simulink model "simscape1j"  (R2025b)
settings: Solver=ode15s  StartTime=0.0  StopTime=100  RelTol=1e-3  AbsTol=1e-3
values from neighbouring files (symbols this model uses):
  g = 32.174    [RCSMasterCalcs.m]    (also in RCS_180_sweep.m)
  Ixxp = 252099.557 * 0.00029263965    (= 73.7743261256)    [ParabolicNozzle.m]    (also in RCSMasterCalcs.m = 54.4132332957; RCS_180_sweep.m = 12.6144279283)
  mdot_slugs = (Cd * A_actual_m2 * P0_Pa * choke / 0.4536) / g    [RCS_180_sweep.m]
  r_nozzle = 5.0 / 12.0    (= 0.416666666667)    [RCS_180_sweep.m]
libraries: fl_lib x18, nesl_utility x8, ee_lib x2
settings Model: Creator=Lana  LastModifiedBy=Lana
settings SolverCC: AutoScaleAbsTol=off  AlgebraicLoopSolver=TrustRegion  MaxZcPerStep=1.0
settings DebuggingCC: UnconnectedInputMsg=warning  UnconnectedOutputMsg=warning  UnconnectedLineMsg=warning  SymbolicDimsDataTypeCodeGenerationDiagnostic=none
settings ModelReferenceCC: EnableRefExpFcnMdlSchedulingChecks=on
settings SFSimCC: CustomCodeUndefinedFunction=UseInterfaceOnly
settings RTWCC: GPUComputeCapability=3.5  DLArmComputeVersion=19.05
settings SimscapeCC: SimscapeLogType=all  SimscapeLogSimulationStatistics=on  SimscapeLogDataHistory=10000.0

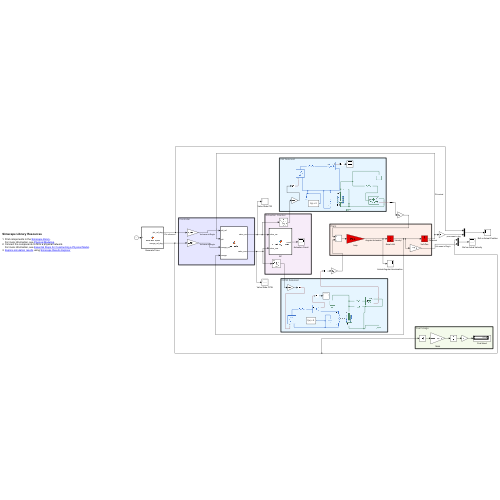
[thumbnail: Simulink's stored preview of the top-level diagram]
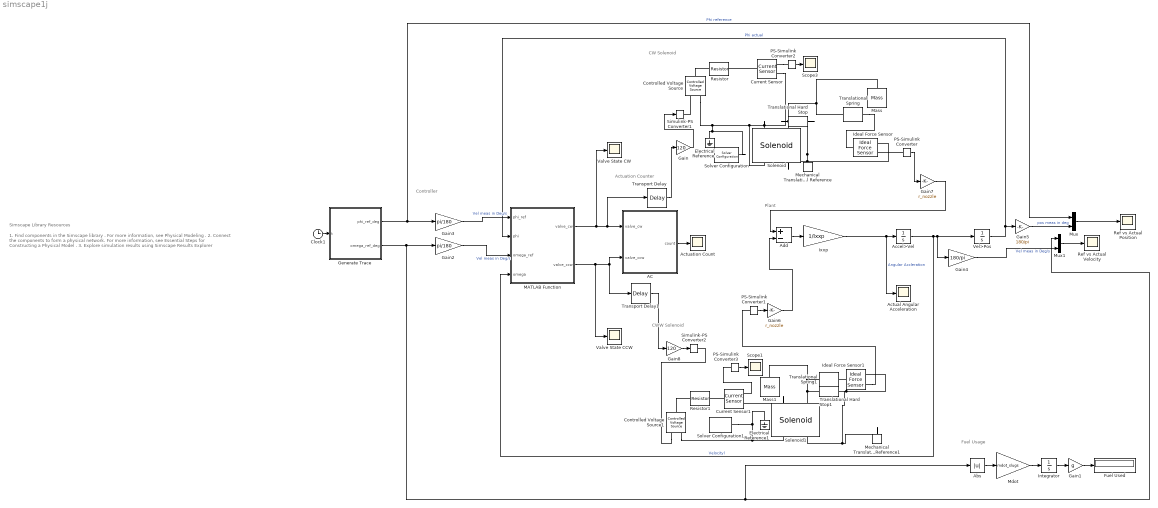
== system simscape1j ==
  note: 1. Find components in the Simscape library .
      | For more information, see Physical Modeling .
      | 2. Connect the components to form a physical network.
      | For more information, see Essential Steps for Constructing a Physical Model .
      | 3. Explore simulation results using Simscape Results Explorer
  note: Simscape Library Resources
  note: Controller
  note: CW Solenoid
  note: Plant
  note: Fuel Usage
  note: Actuation Counter
  note: CWW Solenoid
  AC : MATLAB Function  TreatAsAtomicUnit=on
  Abs : Abs  SaturateOnIntegerOverflow=off
  Accel>Vel : Integrator
  "Actual Angular Acceleration " : Scope
      settings: ActiveDisplayYMinimum=-10.034483776335616  ActiveDisplayYMaximum=37.904655593220141  DataLoggingVariableName=ScopeData4
  Actuation Count : Scope
      settings: ActiveDisplayYMinimum=-1.4453272832049562  ActiveDisplayYMaximum=5.9313739118884694  DataLoggingVariableName=ScopeData3
  Add : Sum  Inputs=+-
  Clock1 : Clock
  Controlled Voltage Source : fl_lib/Electrical/Electrical Sources/Controlled Voltage Source
  Controlled Voltage Source1 : fl_lib/Electrical/Electrical Sources/Controlled Voltage Source
  Current Sensor : fl_lib/Electrical/Electrical Sensors/Current Sensor
  Current Sensor1 : fl_lib/Electrical/Electrical Sensors/Current Sensor
  Electrical Reference : fl_lib/Electrical/Electrical Elements/Electrical Reference
  Electrical Reference1 : fl_lib/Electrical/Electrical Elements/Electrical Reference
  Fuel Used : Display
  Gain : Gain  Gain=120
  Gain1 : Gain  Gain=g
  Gain2 : Gain  Gain=pi/180
  Gain3 : Gain  Gain=pi/180
  Gain4 : Gain  Gain=180/pi
  Gain5 : Gain  Gain=180/pi
  Gain6 : Gain  Gain=r_nozzle
  Gain7 : Gain  Gain=r_nozzle
  Gain8 : Gain  Gain=120
  Generate Trace : MATLAB Function  TreatAsAtomicUnit=on
  Ideal Force Sensor : fl_lib/Mechanical/Mechanical Sensors/Ideal Force Sensor
  Ideal Force Sensor1 : fl_lib/Mechanical/Mechanical Sensors/Ideal Force Sensor
  Integrator : Integrator
  Ixxp : Gain  Gain=1/Ixxp
  MATLAB Function : MATLAB Function  TreatAsAtomicUnit=on  SystemSampleTime=0.005
  Mass : fl_lib/Mechanical/Translational Elements/Mass  mass=0.05 kg  num_ports=foundation.enum.numPorts2.one  v_specify=off  v_priority=High  v=0 m/s  v_nominal_specify=off  v_nominal_value=1  v_nominal_unit=m/s  f_specify=off  f_priority=None  f=0 N  f_nominal_specify=off  f_nominal_value=1  f_nominal_unit=N
  Mass1 : fl_lib/Mechanical/Translational Elements/Mass  mass=0.05 kg  num_ports=foundation.enum.numPorts2.one  v_specify=off  v_priority=High  v=0 m/s  v_nominal_specify=off  v_nominal_value=1  v_nominal_unit=m/s  f_specify=off  f_priority=None  f=0 N  f_nominal_specify=off  f_nominal_value=1  f_nominal_unit=N
  Mdot : Gain  Gain=mdot_slugs
  Mechanical Translational Reference : fl_lib/Mechanical/Translational Elements/Mechanical Translational Reference
  Mechanical Translational Reference1 : fl_lib/Mechanical/Translational Elements/Mechanical Translational Reference
  Mux : Mux  Inputs=2
  Mux1 : Mux  Inputs=2
  PS-Simulink Converter{,1..3} (4 alike) : nesl_utility/PS-Simulink Converter  PhysicalDomain=network_engine_domain  SubClassName=ps_output  LeftPortType=input  RightPortType=output  PseudoPeriodic=off  Frequencies=[]  VectorFormat=inherit  Unit=inherit  AffineConversion=off
  Ref vs Actual Position : Scope
      settings: ActiveDisplayYMinimum=-22.500002652240926  ActiveDisplayYMaximum=202.50000029469345  DataLoggingVariableName=ScopeData5
  Ref vs Actual Velocity : Scope
      settings: ActiveDisplayYMinimum=-4.4232598731139454  ActiveDisplayYMaximum=10.223921060317231
  Resistor : fl_lib/Electrical/Electrical Elements/Resistor  R=1200 Ohm  i_specify=off  i_priority=None  i=0 A  i_nominal_specify=off  i_nominal_value=1  i_nominal_unit=A  v_specify=off  v_priority=None  v=0 V  v_nominal_specify=off  v_nominal_value=1  v_nominal_unit=V
  Resistor1 : fl_lib/Electrical/Electrical Elements/Resistor  R=1200 Ohm  i_specify=off  i_priority=None  i=0 A  i_nominal_specify=off  i_nominal_value=1  i_nominal_unit=A  v_specify=off  v_priority=None  v=0 V  v_nominal_specify=off  v_nominal_value=1  v_nominal_unit=V
  Scope1 : Scope
      settings: ActiveDisplayYMinimum=-0.01250008529219436  ActiveDisplayYMaximum=0.11250076762974927  DataLoggingVariableName=ScopeData2
  Scope3 : Scope
      settings: ActiveDisplayYMinimum=-0.01250008529219436  ActiveDisplayYMaximum=0.11250076762974927  DataLoggingVariableName=ScopeData8
  Simulink-PS Converter1 : nesl_utility/Simulink-PS Converter  PhysicalDomain=network_engine_domain  SubClassName=ps_input  LeftPortType=input  RightPortType=output  PseudoPeriodic=off  Frequencies=[]  NoiseDistribution=none  NoiseParameters=[]  Unit=1  AffineConversion=off  FilteringAndDerivatives=filter  SimscapeFilterOrder=1  InputFilterTimeConstant=0.001  UdotUserProvided=0
  Simulink-PS Converter2 : nesl_utility/Simulink-PS Converter  PhysicalDomain=network_engine_domain  SubClassName=ps_input  LeftPortType=input  RightPortType=output  PseudoPeriodic=off  Frequencies=[]  NoiseDistribution=none  NoiseParameters=[]  Unit=1  AffineConversion=off  FilteringAndDerivatives=filter  SimscapeFilterOrder=1  InputFilterTimeConstant=0.001  UdotUserProvided=0
  Solenoid : ee_lib/Electromechanical/Mechatronic Actuators/Solenoid  motionDirection=ee.enum.actuators.solenoidDirection.towards  F12=[100, 45] N  X12=[0.1, 1.5] mm  Vdc=120 V  Imax=0.133 A  K=25000 N/m  Xzero=0 mm  lam=50 N*s/m  Mass=0.08 kg  Xmax=5 mm  K_endstop=1e8 N/m  D_endstop=500 N*s/m  i_specify=on  i_priority=Low  i=0 A  i_nominal_specify=off  i_nominal_value=0.1  i_nominal_unit=A  x_specify=on  x_priority=Low  x=0.1 mm  x_nominal_specify=off  x_nominal_value=1  x_nominal_unit=mm  vel_specify=on  vel_priority=High  vel=0 mm/s  vel_nominal_specify=off  vel_nominal_value=1  vel_nominal_unit=mm/s  F_specify=on  F_priority=High  F=0 N  F_nominal_specify=off  F_nominal_value=100  F_nominal_unit=N  v_L_specify=off  v_L_priority=None  v_L=0 V  v_L_nominal_specify=off  v_L_nominal_value=1  v_L_nominal_unit=V  magnetic_force_specify=off  magnetic_force_priority=None  magnetic_force=0 N  magnetic_force_nominal_specify=off  magnetic_force_nominal_value=1  magnetic_force_nominal_unit=N  alpha=3.93e-3 1/K  Tmeas=25 degC  thermal_mass=100 J/K  temperature_specify=off  temperature_priority=High  temperature=25 degC  temperature_nominal_specify=off  temperature_nominal_value=1  temperature_nominal_unit=degC  Q_specify=off  Q_priority=None  Q=0 W  Q_nominal_specify=off  Q_nominal_value=1  Q_nominal_unit=W
      settings: InternalSimscapePortConfiguration="{\"Bottom\":[],\"Left\":[{\"id\":\"p\",\"label\":\"+\",\"type\":\"foundation.electrical.electrical\"},{\"id\":\"R\",\"label\":\"R\",\"type\":\"foundation.mechanical.translational.translational\"}],\"Right\":[{\"id\":\"n\",\"label\":\"-\",\"type\":\"foundation.electrical.electrical\"},{\"id\":\"C\",\"label\":\"C\",\"type\":\"foundation.mechanical.translational.translational\"}],\"Top\":[]}"
  Solenoid1 : ee_lib/Electromechanical/Mechatronic Actuators/Solenoid  motionDirection=ee.enum.actuators.solenoidDirection.towards  F12=[100, 45] N  X12=[0.1, 1.5] mm  Vdc=120 V  Imax=0.133 A  K=25000 N/m  Xzero=0 mm  lam=50 N*s/m  Mass=0.08 kg  Xmax=5 mm  K_endstop=1e8 N/m  D_endstop=500 N*s/m  i_specify=on  i_priority=Low  i=0 A  i_nominal_specify=off  i_nominal_value=1  i_nominal_unit=A  x_specify=on  x_priority=Low  x=0.1 mm  x_nominal_specify=off  x_nominal_value=1  x_nominal_unit=mm  vel_specify=on  vel_priority=High  vel=0 mm/s  vel_nominal_specify=off  vel_nominal_value=1  vel_nominal_unit=mm/s  F_specify=on  F_priority=High  F=0 N  F_nominal_specify=off  F_nominal_value=1  F_nominal_unit=N  v_L_specify=off  v_L_priority=None  v_L=0 V  v_L_nominal_specify=off  v_L_nominal_value=1  v_L_nominal_unit=V  magnetic_force_specify=off  magnetic_force_priority=None  magnetic_force=0 N  magnetic_force_nominal_specify=off  magnetic_force_nominal_value=1  magnetic_force_nominal_unit=N  alpha=3.93e-3 1/K  Tmeas=25 degC  thermal_mass=100 J/K  temperature_specify=off  temperature_priority=High  temperature=25 degC  temperature_nominal_specify=off  temperature_nominal_value=1  temperature_nominal_unit=degC  Q_specify=off  Q_priority=None  Q=0 W  Q_nominal_specify=off  Q_nominal_value=1  Q_nominal_unit=W
      settings: InternalSimscapePortConfiguration="{\"Bottom\":[],\"Left\":[{\"id\":\"p\",\"label\":\"+\",\"type\":\"foundation.electrical.electrical\"},{\"id\":\"R\",\"label\":\"R\",\"type\":\"foundation.mechanical.translational.translational\"}],\"Right\":[{\"id\":\"n\",\"label\":\"-\",\"type\":\"foundation.electrical.electrical\"},{\"id\":\"C\",\"label\":\"C\",\"type\":\"foundation.mechanical.translational.translational\"}],\"Top\":[]}"
  Solver Configuration : nesl_utility/Solver Configuration  PhysicalDomain=network_engine_domain  SubClassName=solver  LeftPortType=input  RightPortType=generic  Tones=[]  Harmonics=[]  SimulateNoise=off  Profile=off  UseLocalSampling=off  EnableSwitchedLinearOptims=on  FrequencyDomain=off  UseCCode=off  RelTol=0.001  AbsTol=0.001  MinStep=1e-09  ToWorkspace=off  RevertToSquareIcSolve=off  NumHomotopyIterations=100  PhasorMode=off  PhasorModeNumHarmonics=1  ConsistencySolver=NEWTON_XTOL_AFTER_FTOL  IndexReductionMethod=DerivativeReplacement  DoDC=off  ResidualTolerance=1e-09  ConsistencyTolSource=GLOBAL  ConsistencyAbsTol=0.001  ConsistencyRelTol=0.001  ConsistencyTolFactor=0.001  UseLocalSolver=off  LocalSolverChoice=NE_BACKWARD_EULER_ADVANCER  ResolveIndetEquations=on  FunctionEvalNumThread=1  LocalSolverSampleTime=0.001  DoFixedCost=off  MaxNonlinIter=3  MaxModeIter=2  ComputeImpulses=off  ImpulseIterations=2  LinearAlgebra=auto  LinearAlgebraNumThread=0  EquationFormulation=NE_TIME_EF  DelaysMemoryBudget=1024  AutomaticFiltering=on  FilteringTimeConstant=0.001  PartitionStorageMethod=AS_NEEDED  PartitionMemoryBudget=1024  PartitionMethod=ROBUST  MultibodyUseLocalSolver=off  MultibodyLocalSolverChoice=ODE1  MultibodyLocalSolverSampleTime=0.001
  Solver Configuration1 : nesl_utility/Solver Configuration  PhysicalDomain=network_engine_domain  SubClassName=solver  LeftPortType=input  RightPortType=generic  Tones=[]  Harmonics=[]  SimulateNoise=off  Profile=off  UseLocalSampling=off  EnableSwitchedLinearOptims=on  FrequencyDomain=off  UseCCode=off  RelTol=0.001  AbsTol=0.001  MinStep=1e-09  ToWorkspace=off  RevertToSquareIcSolve=off  NumHomotopyIterations=100  PhasorMode=off  PhasorModeNumHarmonics=1  ConsistencySolver=NEWTON_XTOL_AFTER_FTOL  IndexReductionMethod=DerivativeReplacement  DoDC=off  ResidualTolerance=1e-09  ConsistencyTolSource=GLOBAL  ConsistencyAbsTol=0.001  ConsistencyRelTol=0.001  ConsistencyTolFactor=0.001  UseLocalSolver=off  LocalSolverChoice=NE_BACKWARD_EULER_ADVANCER  ResolveIndetEquations=on  FunctionEvalNumThread=1  LocalSolverSampleTime=0.001  DoFixedCost=off  MaxNonlinIter=3  MaxModeIter=2  ComputeImpulses=off  ImpulseIterations=2  LinearAlgebra=auto  LinearAlgebraNumThread=0  EquationFormulation=NE_TIME_EF  DelaysMemoryBudget=1024  AutomaticFiltering=on  FilteringTimeConstant=0.001  PartitionStorageMethod=AS_NEEDED  PartitionMemoryBudget=1024  PartitionMethod=ROBUST  MultibodyUseLocalSolver=off  MultibodyLocalSolverChoice=ODE1  MultibodyLocalSolverSampleTime=0.001
  Translational Hard Stop : fl_lib/Mechanical/Translational Elements/Translational Hard Stop  upper_bnd=0.005 m  lower_bnd=-.0001 m  model=simscape.enum.hardstop.smooth  stiff_up=1e6 N/m  stiff_low=1e6 N/m  D_up=150 N*s/m  D_low=150 N*s/m  transition=0.1 mm  coeff_rest=0.7  v_tol=0.001 m/s  f_tol=0.001 N  v_specify=off  v_priority=None  v=0 m/s  v_nominal_specify=off  v_nominal_value=1  v_nominal_unit=m/s  f_specify=off  f_priority=None  f=0 N  f_nominal_specify=off  f_nominal_value=1  f_nominal_unit=N  x_specify=off  x_priority=High  x=0 m  x_nominal_specify=off  x_nominal_value=1  x_nominal_unit=m  M_specify=off  M_priority=None  M=0
  Translational Hard Stop1 : fl_lib/Mechanical/Translational Elements/Translational Hard Stop  upper_bnd=0.005 m  lower_bnd=-.0001 m  model=simscape.enum.hardstop.smooth  stiff_up=1e6 N/m  stiff_low=1e6 N/m  D_up=150 N*s/m  D_low=150 N*s/m  transition=0.1 mm  coeff_rest=0.7  v_tol=0.001 m/s  f_tol=0.001 N  v_specify=off  v_priority=None  v=0 m/s  v_nominal_specify=off  v_nominal_value=1  v_nominal_unit=m/s  f_specify=off  f_priority=None  f=0 N  f_nominal_specify=off  f_nominal_value=1  f_nominal_unit=N  x_specify=off  x_priority=High  x=0 m  x_nominal_specify=off  x_nominal_value=1  x_nominal_unit=m  M_specify=off  M_priority=None  M=0
  Translational Spring : fl_lib/Mechanical/Translational Elements/Translational Spring  spr_rate=1000 N/m  v_specify=off  v_priority=None  v=0 m/s  v_nominal_specify=off  v_nominal_value=1  v_nominal_unit=m/s  f_specify=off  f_priority=None  f=0 N  f_nominal_specify=off  f_nominal_value=1  f_nominal_unit=N  x_specify=on  x_priority=High  x=0 m  x_nominal_specify=off  x_nominal_value=1  x_nominal_unit=m
  Translational Spring1 : fl_lib/Mechanical/Translational Elements/Translational Spring  spr_rate=1000 N/m  v_specify=off  v_priority=None  v=0 m/s  v_nominal_specify=off  v_nominal_value=1  v_nominal_unit=m/s  f_specify=off  f_priority=None  f=0 N  f_nominal_specify=off  f_nominal_value=1  f_nominal_unit=N  x_specify=on  x_priority=High  x=0 m  x_nominal_specify=off  x_nominal_value=1  x_nominal_unit=m
  Transport Delay : TransportDelay  DelayTime=0.005
  Transport Delay1 : TransportDelay  DelayTime=0.005
  Valve State CCW : Scope
      settings: ActiveDisplayYMinimum=-9.4532754541059649  ActiveDisplayYMaximum=24.111436479997359
  Valve State CW : Scope
      settings: ActiveDisplayYMinimum=-6.29168187284065  ActiveDisplayYMaximum=5.2016376361109637  DataLoggingVariableName=ScopeData6
  Vel>Pos : Integrator
  wires:
  Abs/1 -> Mdot/1
  Mux/1 -> Ref vs Actual Position/1
  Gain4/1 -> Mux1/2  "Vel meas in Deg/s"
  MATLAB Function/1(valve_cw) -> Valve State CW/1, AC/1(valve_cw), Transport Delay/1
  Transport Delay/1 -> Gain/1
  Gain5/1 -> Mux/2  "pos meas in deg"
  Integrator/1 -> Gain1/1
  Ixxp/1 -> Accel>Vel/1, "Actual Angular Acceleration "/1  "Angular Accleration"
  Mux1/1 -> Ref vs Actual Velocity/1
  Clock1/1 -> Generate Trace/1(t)
  Gain1/1 -> Fuel Used/1
  Vel>Pos/1 -> Gain5/1, MATLAB Function/2(phi)  "Phi actual"
  Mdot/1 -> Integrator/1
  Accel>Vel/1 -> Vel>Pos/1, Gain4/1, MATLAB Function/4(omega)  "Velocityl"
  MATLAB Function/2(valve_ccw) -> AC/2(valve_ccw), Transport Delay1/1, Valve State CCW/1
  Transport Delay1/1 -> Gain8/1
  Gain7/1 -> Add/1
  Gain6/1 -> Add/2
  PS-Simulink Converter/1 -> Gain7/1
  PS-Simulink Converter1/1 -> Gain6/1
  Add/1 -> Ixxp/1
  Gain8/1 -> Simulink-PS Converter2/1
  Generate Trace/2(omega_ref_deg) -> Abs/1, Mux1/1, Gain2/1
  Gain3/1 -> MATLAB Function/1(phi_ref)  "Vel meas in Deg/s"
  Gain2/1 -> MATLAB Function/3(omega_ref)  "Vel meas in Deg/s"
  Generate Trace/1(phi_ref_deg) -> Mux/1, Gain3/1  "Phi reference"
  AC/1(count) -> Actuation Count/1
  Gain/1 -> Simulink-PS Converter1/1
  PS-Simulink Converter2/1 -> Scope3/1
  PS-Simulink Converter3/1 -> Scope1/1
  connections:
  Simulink-PS Converter1/RConn1 -- Controlled Voltage Source/RConn1
  Solenoid/RConn2 -- Translational Hard Stop/RConn1 -- Mechanical Translational Reference/LConn1 -- Ideal Force Sensor/RConn1
  PS-Simulink Converter/LConn1 -- Ideal Force Sensor/RConn2
  Mechanical Translational Reference1/LConn1 -- Solenoid1/RConn2 -- Translational Hard Stop1/RConn1 -- Ideal Force Sensor1/RConn1
  Translational Spring1/RConn1 -- Ideal Force Sensor1/LConn1
  Electrical Reference1/LConn1 -- Solenoid1/RConn1 -- Controlled Voltage Source1/RConn2 -- Solver Configuration1/RConn1
  Controlled Voltage Source1/RConn1 -- Simulink-PS Converter2/RConn1
  Translational Spring1/LConn1 -- Mass1/LConn1 -- Solenoid1/LConn2 -- Translational Hard Stop1/LConn1
  Ideal Force Sensor1/RConn2 -- PS-Simulink Converter1/LConn1
  Controlled Voltage Source/RConn2 -- Electrical Reference/LConn1 -- Solver Configuration/RConn1 -- Solenoid/LConn1 -- Current Sensor/RConn2 -- Solenoid/RConn1
  Translational Spring/RConn1 -- Ideal Force Sensor/LConn1
  Solenoid/LConn2 -- Translational Spring/LConn1 -- Mass/LConn1 -- Translational Hard Stop/LConn1
  Controlled Voltage Source/LConn1 -- Resistor/LConn1
  Resistor1/LConn1 -- Controlled Voltage Source1/LConn1
  Current Sensor/LConn1 -- Resistor/RConn1
  Current Sensor/RConn1 -- PS-Simulink Converter2/LConn1
  Current Sensor1/LConn1 -- Resistor1/RConn1
  Solenoid1/LConn1 -- Current Sensor1/RConn2
  PS-Simulink Converter3/LConn1 -- Current Sensor1/RConn1

== matlab function simscape1j/Generate Trace ==
  data: t input; phi_ref_deg output; omega_ref_deg output
function [phi_ref_deg, omega_ref_deg] = generate_trace(t)
    start_time = 1.0;
    duration = 10.0;
    target_angle = 180.0;
    
    if t < start_time
        phi_ref_deg = 0;
        omega_ref_deg = 0;
    elseif t <= (start_time + duration)
        % Normalized maneuver time (0 to 1)
        tau = (t - start_time) / duration;
        
        % Smooth 5th-order S-curve trajectory
        phi_ref_deg = target_angle * (10*tau^3 - 15*tau^4 + 6*tau^5);
        omega_ref_deg = (target_angle / duration) * (30*tau^2 - 60*tau^3 + 30*tau^4);
    else
        phi_ref_deg = target_angle;
        omega_ref_deg = 0;
    end
end

== matlab function simscape1j/MATLAB Function ==
  settings: updateMethod=DISCRETE
  data: phi_ref input; valve_cw output; valve_ccw output; phi input; omega_ref input; omega input
function [valve_cw, valve_ccw] = rcs_logic(phi_ref, phi, omega_ref, omega)
% Schmitt-trigger valve logic with minimum pulse time.
% Matches RCS_180_sweep.m exactly.
%
% Inputs:
%   phi_ref   - target angle (rad)
%   phi       - actual angle (rad)
%   omega_ref - target angular rate (rad/s)
%   omega     - actual angular rate (rad/s)
% Outputs:
%   valve_cw  - 1 when the clockwise thruster should fire, else 0
%   valve_ccw - 1 when the counter-clockwise thruster should fire, else 0

    % persistent variables keep their value between time steps
    persistent valve_state pulse_timer

    % first time this runs, initialize everything to zero
    if isempty(valve_state)
        valve_state  = 0;
        pulse_timer  = 0;
    end

    % --- Controller gains (match the script) ---
    Kp = 2;
    Kd = 5;

    % --- Schmitt trigger parameters (match the script) ---
    deadzone       = 0.02;
    hysteresis     = 0.01;
    min_pulse_time = 0.10;
    dt             = 0.005;   % must match this block's fixed sample time

    % --- PD control effort ---
    error_phi     = phi_ref - phi;
    error_omega   = omega_ref - omega;
    control_effort = (Kp * error_phi) + (Kd * error_omega);

    % --- Minimum pulse timer countdown ---
    if pulse_timer > 0
        pulse_timer = pulse_timer - dt;

    else
        % --- Schmitt trigger state machine ---
        if valve_state == 0
            if control_effort > deadzone
                valve_state = 1;
                pulse_timer = min_pulse_time;
            elseif control_effort < -deadzone
                valve_state = -1;
                pulse_timer = min_pulse_time;
            end

        elseif valve_state == 1
            if control_effort < (deadzone - hysteresis)
                valve_state = 0;
            end

        elseif valve_state == -1
            if control_effort > -(deadzone - hysteresis)
                valve_state = 0;
            end
        end
    end

    % --- Convert signed valve_state into two separate 0/1 outputs ---
    valve_cw  = double(valve_state == 1);
    valve_ccw = double(valve_state == -1);

end

== matlab function simscape1j/AC ==
  data: valve_cw input; count output; valve_ccw input
function count = actuation_counter(valve_cw, valve_ccw)
% Counts a "firing" each time a thruster turns ON from OFF.
% Inputs:
%   valve_cw  - 1 when the clockwise thruster is firing, else 0
%   valve_ccw - 1 when the counter-clockwise thruster is firing, else 0
% Output:
%   count - running total of firings so far

    % persistent variables keep their value between time steps
    persistent total prev_cw prev_ccw

    % first time this runs, initialize everything to zero
    if isempty(total)
        total   = 0;
        prev_cw  = 0;
        prev_ccw = 0;
    end

    % a "firing" is a transition from 0 -> 1 on either valve
    cw_just_turned_on  = (valve_cw  == 1) && (prev_cw  == 0);
    ccw_just_turned_on = (valve_ccw == 1) && (prev_ccw == 0);

    if cw_just_turned_on || ccw_just_turned_on
        total = total + 1;
    end

    % remember this step's values for next time
    prev_cw  = valve_cw;
    prev_ccw = valve_ccw;

    count = total;
end
